simulink model "Guardian_Top_session_for_integrated"  (R2025b)
settings: Solver=FixedStepAuto  StartTime=0.0  StopTime=100  FixedStep=0.1  RelTol=1e-3
model workspace (MAT data in the model file):
  front_gain_calibration = 0.566985628904
  left_gain_calibration = 0.66316
  right_gain_calibration = 1.44199785177
settings Model: Creator=Ahmed  LastModifiedBy=LENOVO

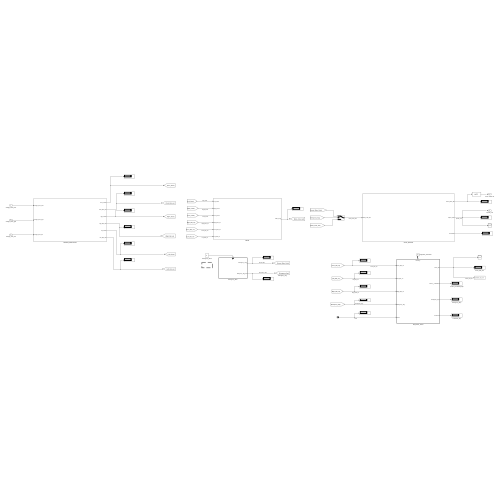
[thumbnail: Simulink's stored preview of the top-level diagram]
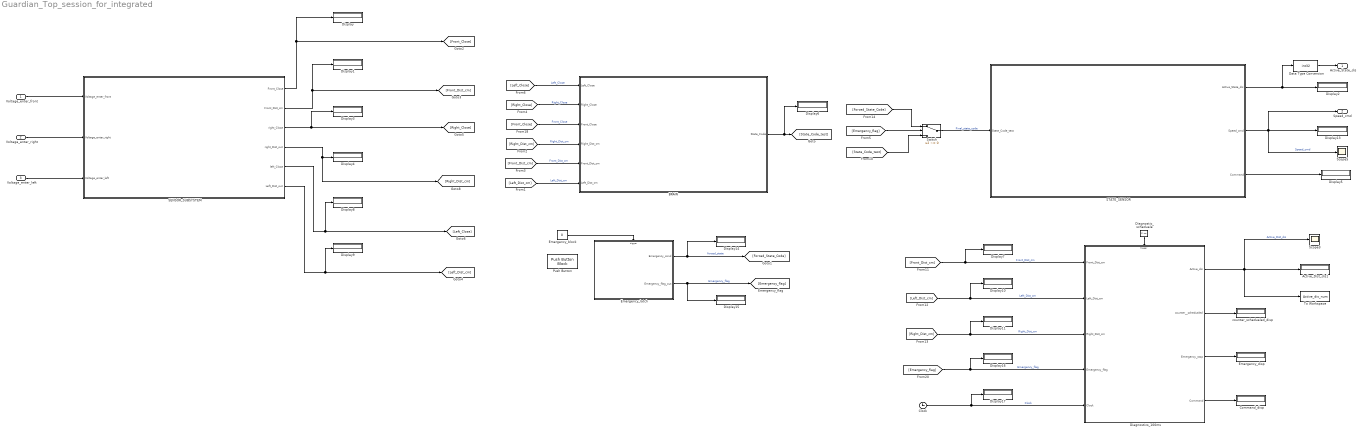
== system Guardian_Top_session_for_integrated ==
  Voltage_enter_front : Inport
  Voltage_enter_right : Inport  Port=2
  Voltage_enter_left : Inport  Port=3
  Active_Dist_dis1 : Display
  BRAIN : Subsystem
  Clock : Clock
  Command_disp : Display
  Data Type Conversion : DataTypeConversion  OutDataTypeStr=int32  SaturateOnIntegerOverflow=off  RndMeth=Floor
  Diagnostic_scheduale : FunctionCallGenerator  SampleTime=0.1
  Diagnostics_100ms : Subsystem  TreatAsAtomicUnit=on
  Display{,1..11,13..17} (17 alike) : Display
  Emergency_block : Constant  Value=0
  Emergency_disp : Display
  Emergency_latch : Subsystem  TreatAsAtomicUnit=on
  Push Button : PushButtonBlock  IconOnColor=[0.0, 0.39215686274509803, 0.0]  IconOffColor=[0.0, 1.0, 0.0]  OffValue=0.000000
  SENSOR_SUBSYSTEM : Subsystem
  STATE_SENSOR : Subsystem
  Scope3 : Scope
      settings: ActiveDisplayYMinimum=-1  ActiveDisplayYMaximum=1  DataLoggingVariableName=ScopeData4
  Scope5 : Scope
      settings: ActiveDisplayYMinimum=90  ActiveDisplayYMaximum=110  DataLoggingVariableName=ScopeData6
  Switch : Switch  Criteria=u2 ~= 0  SaturateOnIntegerOverflow=off  InputSameDT=off
  To Workspace : ToWorkspace  VariableName=Active_dis_num  SaveFormat=Structure With Time  SampleTime=-1
  counter_schedualed_disp : Display
  Active_State_dis : Outport
  Speed_cmd : Outport  Port=2
  wires:
  STATE_SENSOR/1(Active_State_dis) -> Display2/1, Data Type Conversion/1
  [Left_Close] -> BRAIN/1(Left_Close)  "Left_Close"
  [Right_Close] -> BRAIN/2(Right_Close)  "Right_Close"
  BRAIN/1(State_Code) -> Display6/1, [State_Code_test]
  [Right_Dist_cm] -> BRAIN/4(Right_Dist_cm)  "Right_Dist_cm"
  [Left_Dist_cm] -> BRAIN/6(Left_Dist_cm)  "Left_Dist_cm"
  [Front_Dist_cm] -> BRAIN/5(Front_Dist_cm)  "Front_Dist_cm"
  STATE_SENSOR/3(Command) -> Display5/1
  STATE_SENSOR/2(Speed_cmd) -> Scope5/1, Speed_cmd/1, Display13/1  "Speed_cmd"
  [State_Code_test] -> Switch/3
  Switch/1 -> STATE_SENSOR/1(State_Code_test)  "Final_state_code"
  [Forced_State_Code] -> Switch/1
  [Emergency_flag] -> Switch/2
  Diagnostics_100ms/2(counter__schedualed) -> counter_schedualed_disp/1
  Diagnostic_scheduale/1 -> Diagnostics_100ms/Trigger
  Diagnostics_100ms/1(Active_dis) -> Scope3/1, Active_Dist_dis1/1, To Workspace/1  "Active_Dist_dis"
  [Right_Dist_cm] -> Display11/1, Diagnostics_100ms/3(Right_Dist_cm)  "Right_Dist_cm"
  [Left_Dist_cm] -> Display10/1, Diagnostics_100ms/2(Left_Dist_cm)  "Left_Dist_cm"
  [Front_Dist_cm] -> Display7/1, Diagnostics_100ms/1(Front_Dist_cm)  "Front_Dist_cm"
  Emergency_block/1 -> Emergency_latch/Trigger
  Emergency_latch/1(Emergency_cond) -> Display14/1, [Forced_State_Code]  "forced_state"
  Emergency_latch/2(Emergency_flag_out) -> Display15/1, [Emergency_flag]  "Emergency_flag"
  [Emergency_flag] -> Diagnostics_100ms/4(Emergency_flag), Display16/1  "Emergency_flag"
  Diagnostics_100ms/3(Emergency_stop) -> Emergency_disp/1
  Clock/1 -> Display17/1, Diagnostics_100ms/5(Clock)  "Clock"
  Diagnostics_100ms/4(Command) -> Command_disp/1
  [Front_Close] -> BRAIN/3(Front_Close)  "Front_Close"
  SENSOR_SUBSYSTEM/5(left_Close) -> Display8/1, [Left_Close]
  SENSOR_SUBSYSTEM/1(Front_Close) -> [Front_Close], Display/1
  SENSOR_SUBSYSTEM/4(right_Dist_out) -> [Right_Dist_cm], Display4/1
  SENSOR_SUBSYSTEM/6(Left_Dist_out) -> [Left_Dist_cm], Display9/1
  SENSOR_SUBSYSTEM/2(Front_Dist_cm) -> [Front_Dist_cm], Display1/1
  SENSOR_SUBSYSTEM/3(right_Close) -> Display3/1, [Right_Close]
  Voltage_enter_front/1 -> SENSOR_SUBSYSTEM/1(Voltage_enter_front)
  Voltage_enter_right/1 -> SENSOR_SUBSYSTEM/2(Voltage_enter_right)
  Voltage_enter_left/1 -> SENSOR_SUBSYSTEM/3(Voltage_enter_left)
  Data Type Conversion/1 -> Active_State_dis/1

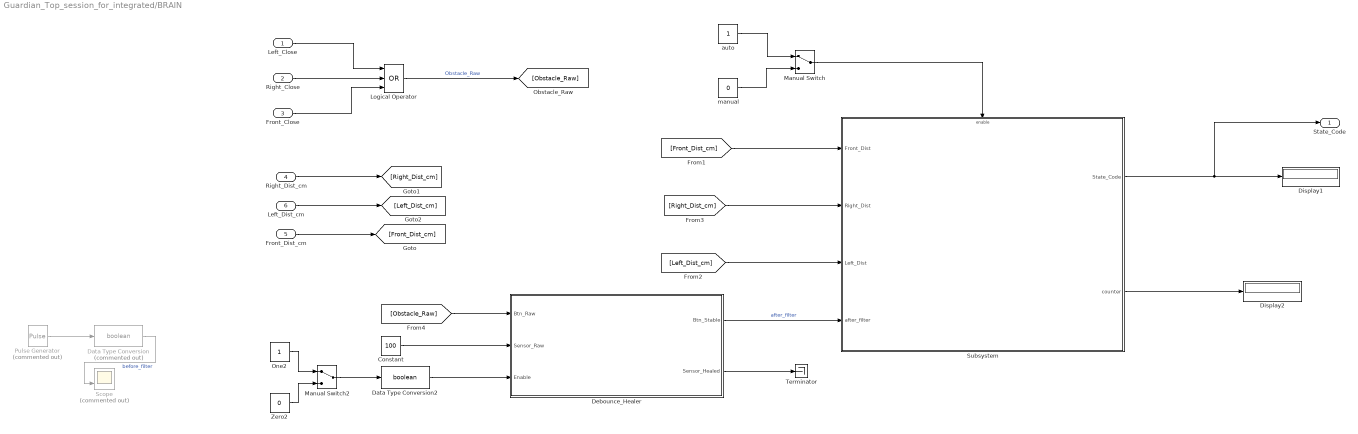
== system Guardian_Top_session_for_integrated/BRAIN ==
  Left_Close : Inport
  Right_Close : Inport  Port=2
  Front_Close : Inport  Port=3
  Right_Dist_cm : Inport  Port=4
  Front_Dist_cm : Inport  Port=5
  Left_Dist_cm : Inport  Port=6
  Constant : Constant  Value=100
  Data Type Conversion : DataTypeConversion  Commented=on  OutDataTypeStr=boolean  SaturateOnIntegerOverflow=off  RndMeth=Floor
  Data Type Conversion2 : DataTypeConversion  OutDataTypeStr=boolean  SaturateOnIntegerOverflow=off  RndMeth=Floor
  Debounce_Healer : Stateflow chart  TreatAsAtomicUnit=on
  Display1 : Display
  Display2 : Display
  Logical Operator : Logic  Operator=OR  Inputs=3  AllPortsSameDT=off  OutDataTypeStr=boolean
  Manual Switch : ManualSwitch
  Manual Switch2 : ManualSwitch
  One2 : Constant  OutDataTypeStr=Inherit: Inherit via back propagation
  Pulse Generator : DiscretePulseGenerator  Commented=on  PulseType=Time based  Period=0.02  PulseWidth=50
  Scope : Scope  Commented=on  NumInputPorts=2
      settings: ActiveDisplayYMinimum=-1  ActiveDisplayYMaximum=1
  Subsystem : Subsystem
  Terminator : Terminator
  Zero2 : Constant  Value=0  OutDataTypeStr=Inherit: Inherit via back propagation
  auto : Constant
  manual : Constant  Value=0
  State_Code : Outport
  wires:
  Logical Operator/1 -> [Obstacle_Raw]  "Obstacle_Raw"
  Right_Close/1 -> Logical Operator/2
  Left_Close/1 -> Logical Operator/1
  Front_Close/1 -> Logical Operator/3
  Left_Dist_cm/1 -> [Left_Dist_cm]
  Right_Dist_cm/1 -> [Right_Dist_cm]
  Front_Dist_cm/1 -> [Front_Dist_cm]
  Data Type Conversion/1 -> Scope/2  "before_filter"
  Pulse Generator/1 -> Data Type Conversion/1
  [Obstacle_Raw] -> Debounce_Healer/1(Btn_Raw)
  Subsystem/1(State_Code) -> State_Code/1, Display1/1
  [Front_Dist_cm] -> Subsystem/1(Front_Dist)
  [Right_Dist_cm] -> Subsystem/2(Right_Dist)
  [Left_Dist_cm] -> Subsystem/3(Left_Dist)
  Debounce_Healer/1(Btn_Stable) -> Subsystem/4(after_filter)  "after_filter"
  Manual Switch/1 -> Subsystem/Enable
  auto/1 -> Manual Switch/1
  manual/1 -> Manual Switch/2
  Subsystem/2(counter) -> Display2/1
  Constant/1 -> Debounce_Healer/2(Sensor_Raw)
  Manual Switch2/1 -> Data Type Conversion2/1
  Data Type Conversion2/1 -> Debounce_Healer/3(Enable)
  One2/1 -> Manual Switch2/1
  Zero2/1 -> Manual Switch2/2
  Debounce_Healer/2(Sensor_Healed) -> Terminator/1

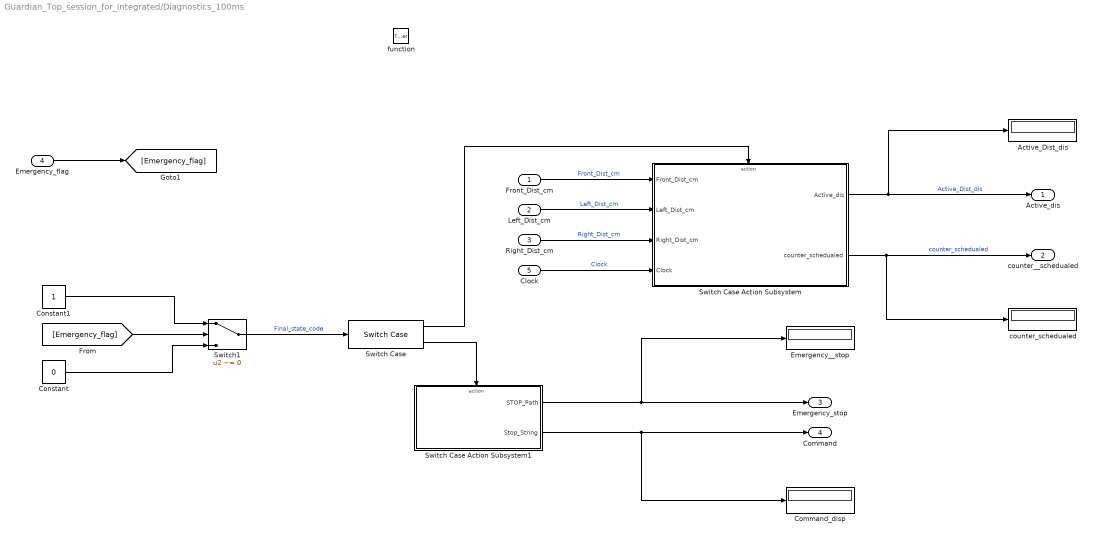
== system Guardian_Top_session_for_integrated/Diagnostics_100ms ==
  Front_Dist_cm : Inport
  Left_Dist_cm : Inport  Port=2
  Right_Dist_cm : Inport  Port=3
  Emergency_flag : Inport  Port=4
  Clock : Inport  Port=5
  function : TriggerPort  TriggerType=function-call  VariantControl=(inherit)
  Active_Dist_dis : Display
  Command_disp : Display
  Constant : Constant  Value=0
  Constant1 : Constant
  Emergency__stop : Display
  Switch Case : SwitchCase  CaseConditions={0 1}  ShowDefaultCase=off
  Switch Case Action Subsystem : Subsystem  TreatAsAtomicUnit=on
  Switch Case Action Subsystem1 : Subsystem  TreatAsAtomicUnit=on
  Switch1 : Switch  Criteria=u2 ~= 0  SaturateOnIntegerOverflow=off  InputSameDT=off
  counter_schedualed : Display
  Active_dis : Outport
  counter__schedualed : Outport  Port=2
  Emergency_stop : Outport  Port=3  OutputWhenDisabled=reset  InitialOutput=0
  Command : Outport  Port=4  OutputWhenDisabled=reset  InitialOutput=0
  wires:
  [Emergency_flag] -> Switch1/2
  Constant1/1 -> Switch1/1
  Emergency_flag/1 -> [Emergency_flag]
  Switch1/1 -> Switch Case/1  "Final_state_code"
  Constant/1 -> Switch1/3
  Switch Case/1 -> Switch Case Action Subsystem/Action
  Switch Case/2 -> Switch Case Action Subsystem1/Action
  Front_Dist_cm/1 -> Switch Case Action Subsystem/1(Front_Dist_cm)  "Front_Dist_cm"
  Left_Dist_cm/1 -> Switch Case Action Subsystem/2(Left_Dist_cm)  "Left_Dist_cm"
  Right_Dist_cm/1 -> Switch Case Action Subsystem/3(Right_Dist_cm)  "Right_Dist_cm"
  Switch Case Action Subsystem/1(Active_dis) -> Active_dis/1, Active_Dist_dis/1  "Active_Dist_dis"
  Switch Case Action Subsystem/2(counter_schedualed) -> counter_schedualed/1, counter__schedualed/1  "counter_schedualed"
  Clock/1 -> Switch Case Action Subsystem/4(Clock)  "Clock"
  Switch Case Action Subsystem1/2(Stop_String) -> Command_disp/1, Command/1
  Switch Case Action Subsystem1/1(STOP_Path) -> Emergency__stop/1, Emergency_stop/1

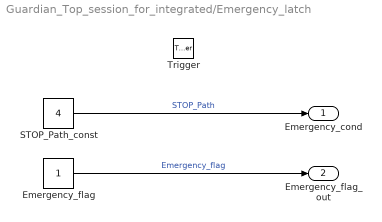
== system Guardian_Top_session_for_integrated/Emergency_latch ==
  Trigger : TriggerPort  VariantControl=(inherit)
  Emergency_flag : Constant
  STOP_Path_const : Constant  Value=4
  Emergency_cond : Outport  InitialOutput=0
  Emergency_flag_out : Outport  Port=2  InitialOutput=0
  wires:
  STOP_Path_const/1 -> Emergency_cond/1  "STOP_Path"
  Emergency_flag/1 -> Emergency_flag_out/1  "Emergency_flag"

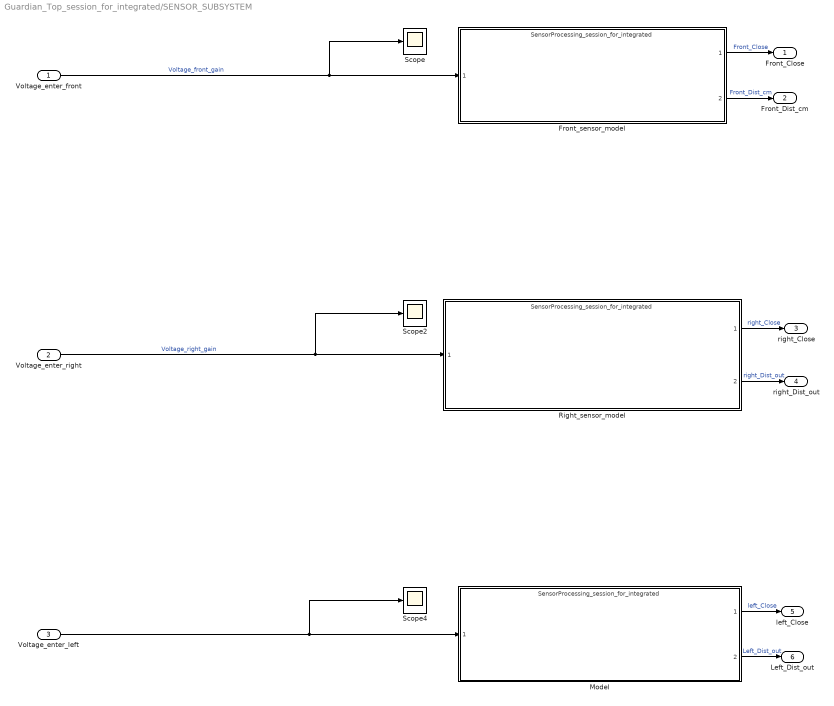
== system Guardian_Top_session_for_integrated/SENSOR_SUBSYSTEM ==
  Voltage_enter_front : Inport
  Voltage_enter_right : Inport  Port=2
  Voltage_enter_left : Inport  Port=3
  Front_sensor_model : ModelReference  ModelNameDialog=SensorProcessing_session_for_integrated.slx  SimulationMode=Normal  ModelReferenceVersion=1.9
  Model : ModelReference  ModelNameDialog=SensorProcessing_session_for_integrated.slx  SimulationMode=Normal  ModelReferenceVersion=1.9
  Right_sensor_model : ModelReference  ModelNameDialog=SensorProcessing_session_for_integrated.slx  SimulationMode=Normal  ModelReferenceVersion=1.9
  Scope : Scope
      settings: ActiveDisplayYMinimum=-0.12499999999999997  ActiveDisplayYMaximum=1.125
  Scope2 : Scope
      settings: ActiveDisplayYMinimum=-0.87499999999999911  ActiveDisplayYMaximum=27.875  DataLoggingVariableName=ScopeData3
  Scope4 : Scope
      settings: ActiveDisplayYMinimum=1.1755399999999998  ActiveDisplayYMaximum=5.42494  DataLoggingVariableName=ScopeData5
  Front_Close : Outport
  Front_Dist_cm : Outport  Port=2
  right_Close : Outport  Port=3
  right_Dist_out : Outport  Port=4
  left_Close : Outport  Port=5
  Left_Dist_out : Outport  Port=6
  wires:
  Voltage_enter_left/1 -> Scope4/1, Model/1
  Front_sensor_model/2 -> Front_Dist_cm/1  "Front_Dist_cm"
  Voltage_enter_front/1 -> Front_sensor_model/1, Scope/1  "Voltage_front_gain"
  Voltage_enter_right/1 -> Right_sensor_model/1, Scope2/1  "Voltage_right_gain"
  Right_sensor_model/1 -> right_Close/1  "right_Close"
  Model/2 -> Left_Dist_out/1  "Left_Dist_out"
  Front_sensor_model/1 -> Front_Close/1  "Front_Close"
  Right_sensor_model/2 -> right_Dist_out/1  "right_Dist_out"
  Model/1 -> left_Close/1  "left_Close"

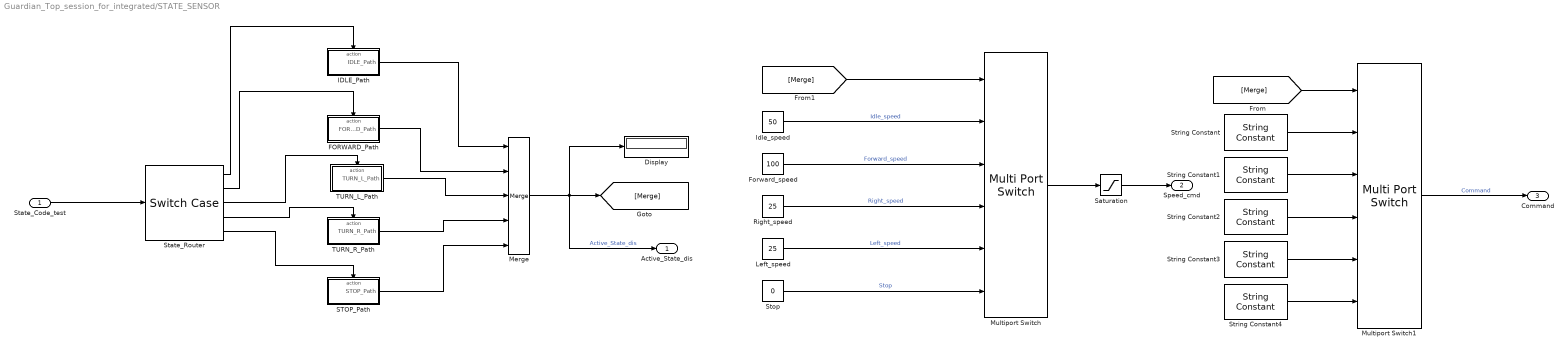
== system Guardian_Top_session_for_integrated/STATE_SENSOR ==
  State_Code_test : Inport
  Display : Display
  FORWARD_Path : Subsystem  TreatAsAtomicUnit=on
  Forward_speed : Constant  Value=100
  IDLE_Path : Subsystem  TreatAsAtomicUnit=on
  Idle_speed : Constant  Value=50
  Left_speed : Constant  Value=25
  Merge : Merge  Inputs=5
  Multiport Switch : MultiPortSwitch  DataPortOrder=Zero-based contiguous  Inputs=5  zeroidx=on  SaturateOnIntegerOverflow=off  InputSameDT=off
  Multiport Switch1 : MultiPortSwitch  DataPortOrder=Zero-based contiguous  Inputs=5  zeroidx=on  SaturateOnIntegerOverflow=off  InputSameDT=off
  Right_speed : Constant  Value=25
  STOP_Path : Subsystem  TreatAsAtomicUnit=on
  Saturation : Saturate  UpperLimit=100  LowerLimit=0
  State_Router : SwitchCase  CaseConditions={0,1,2,3,4}  ShowDefaultCase=off
  Stop : Constant  Value=0
  String Constant : StringConstant  String="\"IDLE Path\""
  String Constant1 : StringConstant  String="\"FORWARD Path\""
  String Constant2 : StringConstant  String="\"TURN Left\""
  String Constant3 : StringConstant  String="\"TURN Right\""
  String Constant4 : StringConstant  String="\"Stop\""
  TURN_L_Path : Subsystem  TreatAsAtomicUnit=on
  TURN_R_Path : Subsystem  TreatAsAtomicUnit=on
  Active_State_dis : Outport
  Speed_cmd : Outport  Port=2
  Command : Outport  Port=3
  wires:
  TURN_R_Path/1(TURN_R_Path) -> Merge/4
  State_Router/2 -> FORWARD_Path/Action
  IDLE_Path/1(IDLE_Path) -> Merge/1
  STOP_Path/1(STOP_Path) -> Merge/5
  FORWARD_Path/1(FORWARD_Path) -> Merge/2
  TURN_L_Path/1(TURN_L_Path) -> Merge/3
  State_Router/4 -> TURN_R_Path/Action
  State_Router/1 -> IDLE_Path/Action
  State_Router/5 -> STOP_Path/Action
  State_Router/3 -> TURN_L_Path/Action
  Merge/1 -> [Merge], Active_State_dis/1, Display/1  "Active_State_dis"
  State_Code_test/1 -> State_Router/1
  String Constant/1 -> Multiport Switch1/2
  Idle_speed/1 -> Multiport Switch/2  "Idle_speed"
  Forward_speed/1 -> Multiport Switch/3  "Forward_speed"
  String Constant3/1 -> Multiport Switch1/5
  Left_speed/1 -> Multiport Switch/5  "Left_speed"
  Saturation/1 -> Speed_cmd/1
  String Constant1/1 -> Multiport Switch1/3
  Stop/1 -> Multiport Switch/6  "Stop"
  Multiport Switch/1 -> Saturation/1
  Right_speed/1 -> Multiport Switch/4  "Right_speed"
  String Constant4/1 -> Multiport Switch1/6
  String Constant2/1 -> Multiport Switch1/4
  Multiport Switch1/1 -> Command/1  "Command"
  [Merge] -> Multiport Switch/1
  [Merge] -> Multiport Switch1/1

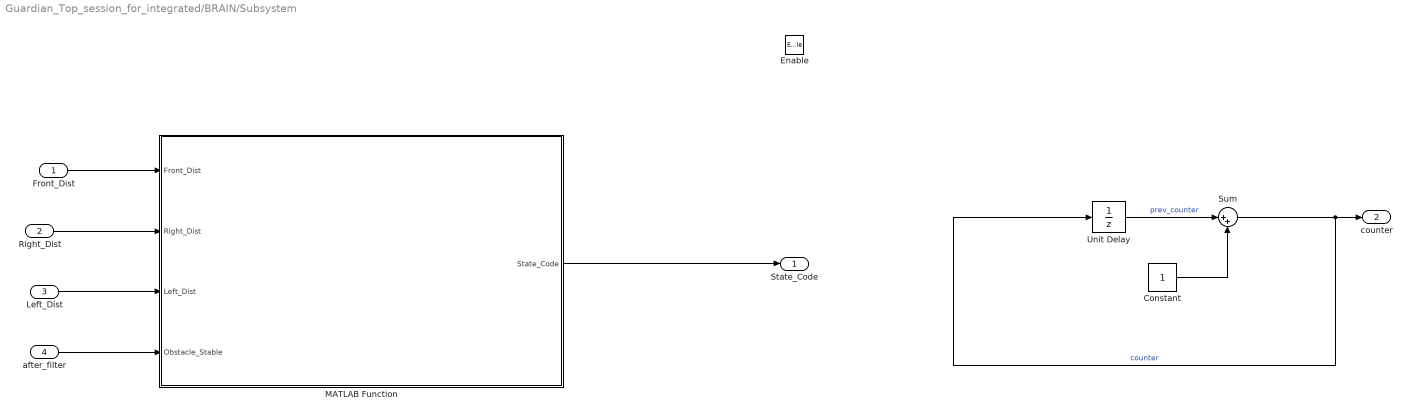
== system Guardian_Top_session_for_integrated/BRAIN/Subsystem ==
  Front_Dist : Inport
  Right_Dist : Inport  Port=2
  Left_Dist : Inport  Port=3
  after_filter : Inport  Port=4
  Enable : EnablePort
  Constant : Constant
  MATLAB Function : MATLAB Function  TreatAsAtomicUnit=on
  Sum : Sum  Inputs=|++
  Unit Delay : UnitDelay  SampleTime=-1  HasFrameUpgradeWarning=on
  State_Code : Outport
  counter : Outport  Port=2
  wires:
  Right_Dist/1 -> MATLAB Function/2(Right_Dist)
  Left_Dist/1 -> MATLAB Function/3(Left_Dist)
  after_filter/1 -> MATLAB Function/4(Obstacle_Stable)
  MATLAB Function/1(State_Code) -> State_Code/1
  Front_Dist/1 -> MATLAB Function/1(Front_Dist)
  Sum/1 -> Unit Delay/1, counter/1  "counter"
  Constant/1 -> Sum/2
  Unit Delay/1 -> Sum/1  "prev_counter"

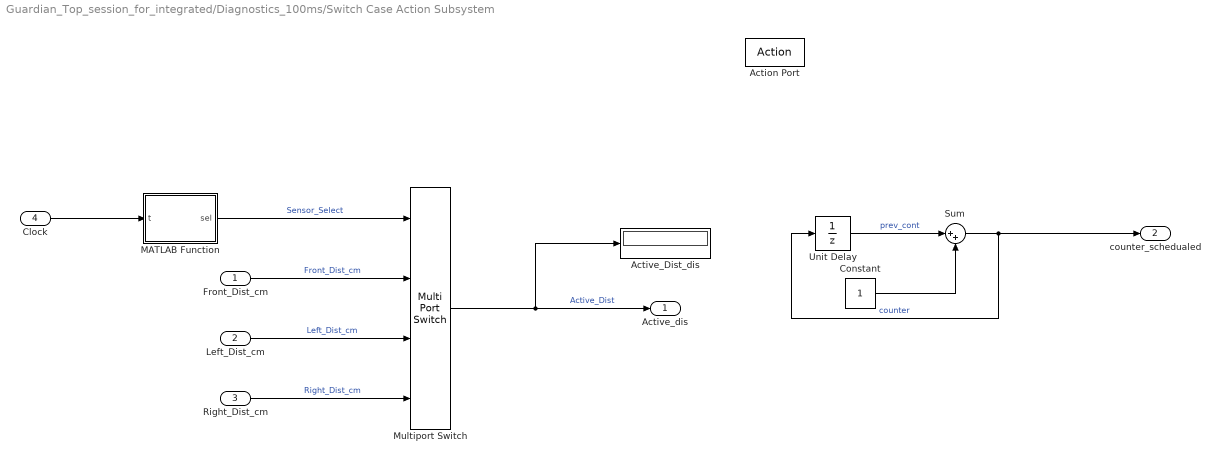
== system Guardian_Top_session_for_integrated/Diagnostics_100ms/Switch Case Action Subsystem ==
  Front_Dist_cm : Inport
  Left_Dist_cm : Inport  Port=2
  Right_Dist_cm : Inport  Port=3
  Clock : Inport  Port=4
  Action Port : ActionPort  ActionPortLabel=case [ 0 ]:
  Active_Dist_dis : Display
  Constant : Constant
  MATLAB Function : MATLAB Function  TreatAsAtomicUnit=on
  Multiport Switch : MultiPortSwitch  SaturateOnIntegerOverflow=off  InputSameDT=off
  Sum : Sum  Inputs=|++
  Unit Delay : UnitDelay  SampleTime=-1  HasFrameUpgradeWarning=on
  Active_dis : Outport
  counter_schedualed : Outport  Port=2
  wires:
  Left_Dist_cm/1 -> Multiport Switch/3  "Left_Dist_cm"
  Front_Dist_cm/1 -> Multiport Switch/2  "Front_Dist_cm"
  MATLAB Function/1(sel) -> Multiport Switch/1  "Sensor_Select"
  Multiport Switch/1 -> Active_Dist_dis/1, Active_dis/1  "Active_Dist"
  Right_Dist_cm/1 -> Multiport Switch/4  "Right_Dist_cm"
  Clock/1 -> MATLAB Function/1(t)
  Unit Delay/1 -> Sum/1  "prev_cont"
  Constant/1 -> Sum/2
  Sum/1 -> Unit Delay/1, counter_schedualed/1  "counter"

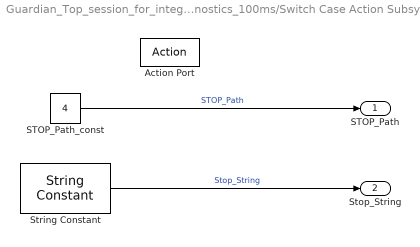
== system Guardian_Top_session_for_integrated/Diagnostics_100ms/Switch Case Action Subsystem1 ==
  Action Port : ActionPort  ActionPortLabel=case [ 1 ]:
  STOP_Path_const : Constant  Value=4
  String Constant : StringConstant  String="\"Stop\""
  STOP_Path : Outport  OutputWhenDisabled=reset  InitialOutput=0
  Stop_String : Outport  Port=2  OutputWhenDisabled=reset  InitialOutput=0
  wires:
  STOP_Path_const/1 -> STOP_Path/1  "STOP_Path"
  String Constant/1 -> Stop_String/1  "Stop_String"

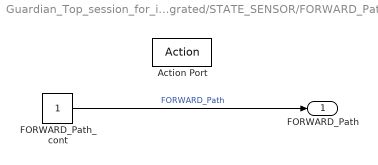
== system Guardian_Top_session_for_integrated/STATE_SENSOR/FORWARD_Path ==
  Action Port : ActionPort  ActionPortLabel=case [ 1 ]:
  FORWARD_Path_cont : Constant
  FORWARD_Path : Outport
  wires:
  FORWARD_Path_cont/1 -> FORWARD_Path/1  "FORWARD_Path"

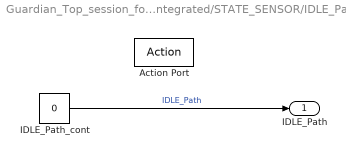
== system Guardian_Top_session_for_integrated/STATE_SENSOR/IDLE_Path ==
  Action Port : ActionPort  ActionPortLabel=case [ 0 ]:
  IDLE_Path_cont : Constant  Value=0
  IDLE_Path : Outport
  wires:
  IDLE_Path_cont/1 -> IDLE_Path/1  "IDLE_Path"

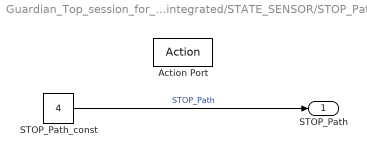
== system Guardian_Top_session_for_integrated/STATE_SENSOR/STOP_Path ==
  Action Port : ActionPort  ActionPortLabel=case [ 4 ]:
  STOP_Path_const : Constant  Value=4
  STOP_Path : Outport
  wires:
  STOP_Path_const/1 -> STOP_Path/1  "STOP_Path"

== system Guardian_Top_session_for_integrated/STATE_SENSOR/TURN_L_Path ==
  Action Port : ActionPort  ActionPortLabel=case [ 2 ]:
  TURN_L_Path_const : Constant  Value=2
  TURN_L_Path : Outport
  wires:
  TURN_L_Path_const/1 -> TURN_L_Path/1  "TURN_L_Path"

== system Guardian_Top_session_for_integrated/STATE_SENSOR/TURN_R_Path ==
  Action Port : ActionPort  ActionPortLabel=case [ 3 ]:
  TURN_R_Path_const : Constant  Value=3
  TURN_R_Path : Outport
  wires:
  TURN_R_Path_const/1 -> TURN_R_Path/1  "TURN_R_Path"

== matlab function Guardian_Top_session_for_integrated/BRAIN/Subsystem/MATLAB Function ==
  data: Front_Dist input; State_Code output; Right_Dist input; Left_Dist input; Obstacle_Stable input
function State_Code  = DecideRobotState(Front_Dist, Right_Dist, Left_Dist, Obstacle_Stable)

    if Obstacle_Stable && Front_Dist < 20
        State_Code = int32(4);
    elseif Obstacle_Stable && Front_Dist < 40 && Left_Dist > Right_Dist
        State_Code = int32(2);
    elseif Obstacle_Stable && Front_Dist < 40
        State_Code = int32(3);
    elseif Front_Dist >= 40
        State_Code = int32(1);
    else
        State_Code = int32(0);
    end
    
end

== matlab function Guardian_Top_session_for_integrated/Diagnostics_100ms/Switch Case Action Subsystem/MATLAB Function ==
  data: t input; sel output
function sel = fcn(t)
    holdTime = 10;        % seconds each value is held
    values   = [1 2 3];  % Front, Left, Right
    idx = mod(floor(t/holdTime), numel(values)) + 1;
    sel = values(idx);
end

== stateflow chart Guardian_Top_session_for_integrated/BRAIN/Debounce_Healer ==
  state ButtonLogic [parallel]
    settings: executionOrder=1
    state Disable
      entry:
      DebounceCounter = 0;
    state Enable
      entry:
      state Off_Stable
        entry:
        Btn_Stable = false;
        du:
        DebounceCounter = 0;
      state On_Stable
        entry:
        Btn_Stable  = true;
        du:
        DebounceCounter = 0;
      (junction 31) -> On_Stable [order 2] : [Btn_Raw == 1] /{DebounceCounter = 0;}
      (default) -> Off_Stable
      On_Stable -> (junction 31) : [Btn_Raw == 0] {DebounceCounter = DebounceCounter + 1;}
      (junction 31) -> Off_Stable [order 1] : [DebounceCounter >= N_confirm] /{DebounceCounter = 0;}
      (junction 31) -> (junction 63) [order 3]
      (junction 60) -> Off_Stable
      (junction 63) -> On_Stable
      (junction 17) -> (junction 60) [order 3]
      Off_Stable -> (junction 17) : [Btn_Raw == 1] {DebounceCounter = DebounceCounter + 1;}
      (junction 17) -> On_Stable [order 1] : [DebounceCounter >= N_confirm] /{DebounceCounter = 0;}
      (junction 17) -> Off_Stable [order 2] : [Btn_Raw == 0] /{DebounceCounter = 0;}
    (default) -> Enable
    Enable -> Disable : [Enable == 0]
    Disable -> (history) : [Enable == 1]
  state SensorLogic [parallel]
    settings: executionOrder=2
    state Trusted
      entry:
      HealCounter = 0;
      du:
      Sensor_Healed = Sensor_Raw;
      LastGood = Sensor_Raw;
    state Healing
      du:
      Sensor_Healed = LastGood;
      HealCounter = 0;
    Healing -> (junction 44) : [Sensor_Raw >= 0 && Sensor_Raw <= 500] {HealCounter = HealCounter + 1;}
    (junction 44) -> Trusted [order 1] : [HealCounter >= N_heal]
    (junction 44) -> (junction 66) [order 3]
    (junction 44) -> Healing [order 2] : [Sensor_Raw < 0 || Sensor_Raw > 500] /{HealCounter = 0;}
    (default) -> Trusted
    (junction 66) -> Healing
    Trusted -> Healing : [Sensor_Raw < 0 || Sensor_Raw > 500]
  (default) -> ButtonLogic
  data: Btn_Raw input boolean; Sensor_Raw input double; Btn_Stable output boolean =0; Sensor_Healed output double =0; DebounceCounter local int32 =0; HealCounter local int32 =0; LastGood local double =0; N_confirm constant double =5; N_heal constant double =10; Enable input boolean
